simulink model "solenoid_valve_curtain_v1_109"  (R2026a)
settings: Solver=ode15s  StopTime=30  AbsTol=1e-3
values from neighbouring files (symbols this model uses):
  g = 32.174    [RCSMasterCalcs.m]    (also in RCS_180_sweep.m)
  Ixxp = 252099.557 * 0.00029263965    (= 73.7743261256)    [ParabolicNozzle.m]    (also in RCSMasterCalcs.m = 54.4132332957; RCS_180_sweep.m = 12.6144279283)
  mdot_slugs = (Cd * A_actual_m2 * P0_Pa * choke / 0.4536) / g    [RCS_180_sweep.m]
  P0_Pa = P0_abs_psi * 6894.76    (= 1480304.972)    [RCSMasterCalcs.m]    (also in RCS_180_sweep.m = P_psi * 6894.76)
  r_nozzle = 5.0 / 12.0    (= 0.416666666667)    [RCS_180_sweep.m]
libraries: fl_lib x14, nesl_utility x8, ee_lib x2
settings Model: Creator=Lana  LastModifiedBy=Yelkan
settings DebuggingCC: SymbolicDimsDataTypeCodeGenerationDiagnostic=none
settings SimscapeCC: SimscapeNominalValues="[{\"value\":\"1\",\"unit\":\"A\"},{\"value\":\"1\",\"unit\":\"bar\"},{\"value\":\"1\",\"unit\":\"cm^2\"},{\"value\":\"1\",\"unit\":\"cm^3/s\"},{\"value\":\"1\",\"unit\":\"kJ/kg\"},{\"value\":\"1\",\"unit\":\"kW\"},{\"value\":\"1\",\"unit\":\"l\"},{\"value\":\"1\",\"unit\":\"N\"},{\"value\":\"1\",\"unit\":\"N*m\"},{\"value\":\"1\",\"unit\":\"V\"}]"  SimscapeLogSimulationStatistics=on

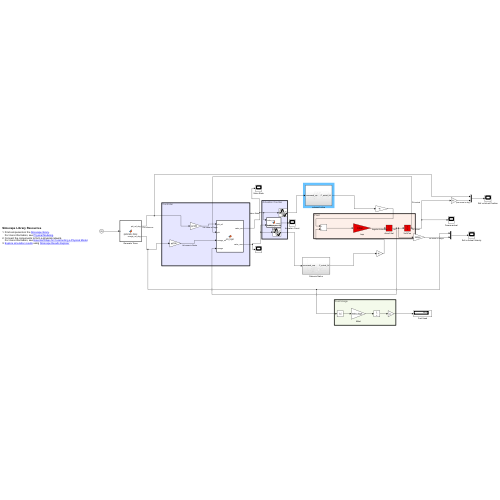
[thumbnail: Simulink's stored preview of the top-level diagram]
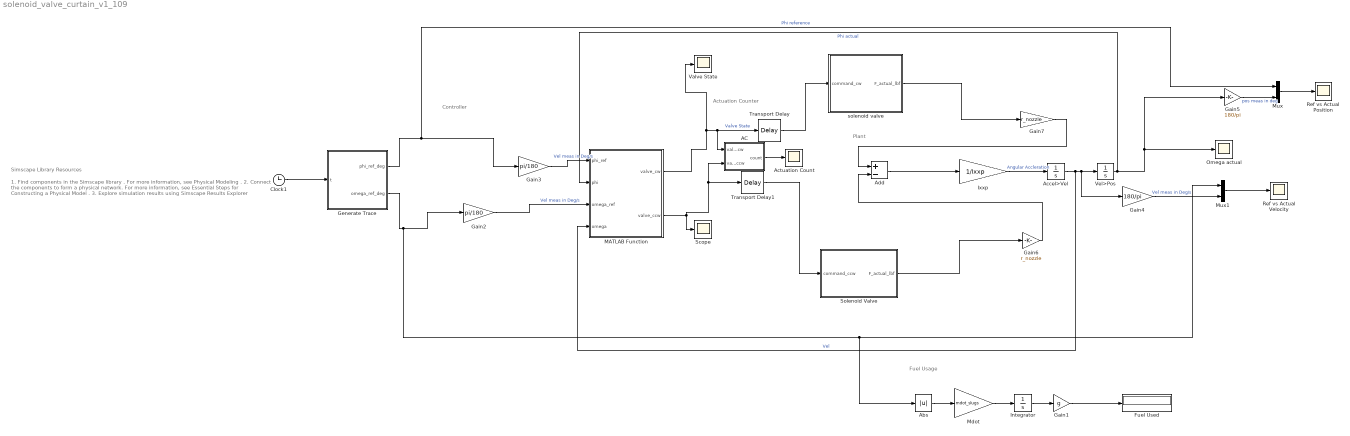
== system solenoid_valve_curtain_v1_109 ==
  note: 1. Find components in the Simscape library .
      | For more information, see Physical Modeling .
      | 2. Connect the components to form a physical network.
      | For more information, see Essential Steps for Constructing a Physical Model .
      | 3. Explore simulation results using Simscape Results Explorer
  note: Simscape Library Resources
  note: Controller
  note: Actuation Counter
  note: Plant
  note: Fuel Usage
  AC : MATLAB Function  TreatAsAtomicUnit=on
  Abs : Abs  SaturateOnIntegerOverflow=off
  Accel>Vel : Integrator
  Actuation Count : Scope
      settings: ActiveDisplayYMinimum=-26.808847302492552  ActiveDisplayYMaximum=50.778884865366138  DataLoggingVariableName=ScopeData3
  Add : Sum  Inputs=+-
  Clock1 : Clock
  Fuel Used : Display
  Gain1 : Gain  Gain=g
  Gain2 : Gain  Gain=pi/180
  Gain3 : Gain  Gain=pi/180
  Gain4 : Gain  Gain=180/pi
  Gain5 : Gain  Gain=180/pi
  Gain6 : Gain  Gain=r_nozzle
  Gain7 : Gain  Gain=r_nozzle
  Generate Trace : MATLAB Function  TreatAsAtomicUnit=on
  Integrator : Integrator
  Ixxp : Gain  Gain=1/Ixxp
  MATLAB Function : MATLAB Function  TreatAsAtomicUnit=on  SystemSampleTime=0.005
  Mdot : Gain  Gain=mdot_slugs
  Mux : Mux  Inputs=2
  Mux1 : Mux  Inputs=2
  Omega actual : Scope
      settings: ActiveDisplayYMinimum=-0.70228346658885066  ActiveDisplayYMaximum=6.3205511992996568  DataLoggingVariableName=ScopeData4
  Ref vs Actual Position : Scope
      settings: ActiveDisplayYMinimum=-60.319230844507317  ActiveDisplayYMaximum=326.94611656087733  DataLoggingVariableName=ScopeData5
  Ref vs Actual Velocity : Scope
      settings: ActiveDisplayYMinimum=-10.640842810110598  ActiveDisplayYMaximum=57.185626811535826
  Scope : Scope
      settings: ActiveDisplayYMinimum=0.21360200383868255  ActiveDisplayYMaximum=1.5917270038386833
  Solenoid Valve : Subsystem
  Transport Delay : TransportDelay  DelayTime=0.005
  Transport Delay1 : TransportDelay  DelayTime=0.005
  Valve State : Scope
      settings: ActiveDisplayYMinimum=-3.9526088666508228  ActiveDisplayYMaximum=5.6960106065109395  DataLoggingVariableName=ScopeData6
  Vel>Pos : Integrator
  solenoid valve : Subsystem
  wires:
  Abs/1 -> Mdot/1
  Mux/1 -> Ref vs Actual Position/1
  Gain4/1 -> Mux1/2  "Vel meas in Deg/s"
  MATLAB Function/1(valve_cw) -> Transport Delay/1, AC/1(valve_cw), Valve State/1  "Valve State"
  Gain5/1 -> Mux/2  "pos meas in deg"
  Integrator/1 -> Gain1/1
  Ixxp/1 -> Accel>Vel/1  "Angular Accleration"
  Mux1/1 -> Ref vs Actual Velocity/1
  Clock1/1 -> Generate Trace/1(t)
  Gain1/1 -> Fuel Used/1
  Vel>Pos/1 -> MATLAB Function/2(phi), Gain5/1, Omega actual/1  "Phi actual"
  Mdot/1 -> Integrator/1
  Accel>Vel/1 -> MATLAB Function/4(omega), Gain4/1, Vel>Pos/1  "Vel"
  MATLAB Function/2(valve_ccw) -> Transport Delay1/1, AC/2(valve_ccw), Scope/1
  Gain7/1 -> Add/1
  Gain6/1 -> Add/2
  Add/1 -> Ixxp/1
  Generate Trace/2(omega_ref_deg) -> Gain2/1, Abs/1, Mux1/1
  Gain3/1 -> MATLAB Function/1(phi_ref)  "Vel meas in Deg/s"
  Gain2/1 -> MATLAB Function/3(omega_ref)  "Vel meas in Deg/s"
  Generate Trace/1(phi_ref_deg) -> Mux/1, Gain3/1  "Phi reference"
  AC/1(count) -> Actuation Count/1
  solenoid valve/1("F_actual_lbf ") -> Gain7/1
  Transport Delay1/1 -> Solenoid Valve/1(command_ccw)
  Solenoid Valve/1(F_actual_lbf) -> Gain6/1
  Transport Delay/1 -> solenoid valve/1("command_cw ")

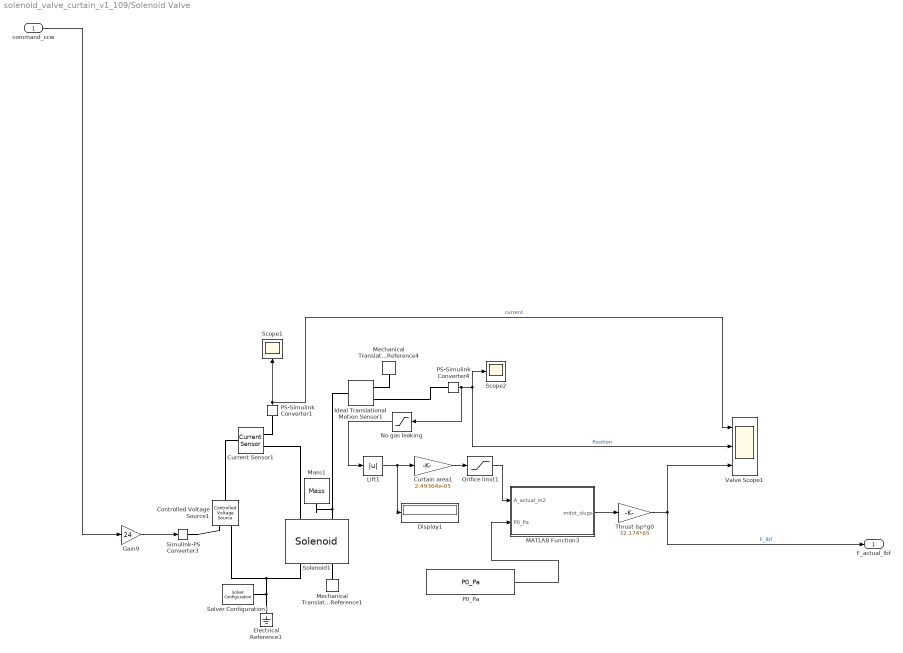
== system solenoid_valve_curtain_v1_109/Solenoid Valve ==
  command_ccw : Inport
  Controlled Voltage Source1 : fl_lib/Electrical/Electrical Sources/Controlled Voltage Source
  Current Sensor1 : fl_lib/Electrical/Electrical Sensors/Current Sensor
  Curtain area1 : Gain  Gain=2.49364e-05
  Display1 : Display
  Electrical Reference1 : fl_lib/Electrical/Electrical Elements/Electrical Reference
  Gain9 : Gain  Gain=24
  Ideal Translational Motion Sensor1 : fl_lib/Mechanical/Mechanical Sensors/Ideal Translational Motion Sensor  reference=foundation.enum.MeasurementReference.difference  acceleration_port=false  velocity_port=false  position_port=true  offset=0 m
  Lift1 : Abs  SaturateOnIntegerOverflow=off
  MATLAB Function3 : MATLAB Function  TreatAsAtomicUnit=on
  Mass1 : fl_lib/Mechanical/Translational Elements/Mass  mass=0.005 kg  num_ports=foundation.enum.numPorts2.one  v_specify=off  v_priority=High  v=0 m/s  v_nominal_specify=off  v_nominal_value=1  v_nominal_unit=m/s  f_specify=off  f_priority=None  f=0 N  f_nominal_specify=off  f_nominal_value=1  f_nominal_unit=N
  Mechanical Translational Reference1 : fl_lib/Mechanical/Translational Elements/Mechanical Translational Reference
  Mechanical Translational Reference4 : fl_lib/Mechanical/Translational Elements/Mechanical Translational Reference
  No gas leaking : Saturate  UpperLimit=0  LowerLimit=-100
  Orifice limit1 : Saturate  UpperLimit=4.94832e-05  LowerLimit=0
  P0_Pa : Constant  Value=P0_Pa
  PS-Simulink Converter1 : nesl_utility/PS-Simulink Converter  PhysicalDomain=network_engine_domain  SubClassName=ps_output  LeftPortType=input  RightPortType=output  PseudoPeriodic=off  Frequencies=[]  VectorFormat=inherit  Unit=A  AffineConversion=off
  PS-Simulink Converter4 : nesl_utility/PS-Simulink Converter  PhysicalDomain=network_engine_domain  SubClassName=ps_output  LeftPortType=input  RightPortType=output  PseudoPeriodic=off  Frequencies=[]  VectorFormat=inherit  Unit=mm  AffineConversion=off
  Scope1 : Scope
      settings: ActiveDisplayYMinimum=-0.033382252757602926  ActiveDisplayYMaximum=0.30044027481842639  DataLoggingVariableName=ScopeData7
  Scope2 : Scope
      settings: ActiveDisplayYMinimum=-7.0487625645709668  ActiveDisplayYMaximum=0.74377868714144668  DataLoggingVariableName=ScopeData10
  Simulink-PS Converter3 : nesl_utility/Simulink-PS Converter  PhysicalDomain=network_engine_domain  SubClassName=ps_input  LeftPortType=input  RightPortType=output  PseudoPeriodic=off  Frequencies=[]  NoiseDistribution=none  NoiseParameters=[]  Unit=V  AffineConversion=off  FilteringAndDerivatives=filter  SimscapeFilterOrder=1  InputFilterTimeConstant=0.001  UdotUserProvided=0
  Solenoid1 : ee_lib/Electromechanical/Mechatronic Actuators/Solenoid  motionDirection=ee.enum.actuators.solenoidDirection.towards  F12=[100, 45] N  X12=[0.1, 1.5] mm  Vdc=24 V  Imax=0.33 A  K=1500 N/m  Xzero=10.3333 mm  lam=5 N*s/m  Mass=0.010 kg  Xmax=7.94 mm  K_endstop=1e6 N/m  D_endstop=500 N*s/m  i_specify=on  i_priority=High  i=0 A  i_nominal_specify=off  i_nominal_value=0.1  i_nominal_unit=A  x_specify=on  x_priority=High  x=7.94 mm  x_nominal_specify=off  x_nominal_value=1  x_nominal_unit=mm  vel_specify=on  vel_priority=Low  vel=0 mm/s  vel_nominal_specify=off  vel_nominal_value=1  vel_nominal_unit=mm/s  F_specify=off  F_priority=High  F=0 N  F_nominal_specify=off  F_nominal_value=100  F_nominal_unit=N  v_L_specify=off  v_L_priority=None  v_L=0 V  v_L_nominal_specify=off  v_L_nominal_value=1  v_L_nominal_unit=V  magnetic_force_specify=off  magnetic_force_priority=None  magnetic_force=0 N  magnetic_force_nominal_specify=off  magnetic_force_nominal_value=1  magnetic_force_nominal_unit=N  alpha=3.93e-3 1/K  Tmeas=25 degC  thermal_mass=100 J/K  temperature_specify=off  temperature_priority=High  temperature=25 degC  temperature_nominal_specify=off  temperature_nominal_value=1  temperature_nominal_unit=degC  Q_specify=off  Q_priority=None  Q=0 W  Q_nominal_specify=off  Q_nominal_value=1  Q_nominal_unit=W
  Solver Configuration1 : nesl_utility/Solver Configuration  PhysicalDomain=network_engine_domain  SubClassName=solver  LeftPortType=input  RightPortType=generic  Tones=[]  Harmonics=[]  SimulateNoise=off  Profile=off  UseLocalSampling=off  EnableSwitchedLinearOptims=on  FrequencyDomain=off  UseCCode=off  RelTol=0.001  AbsTol=0.001  MinStep=1e-09  ToWorkspace=off  RevertToSquareIcSolve=off  NumHomotopyIterations=100  PhasorMode=off  PhasorModeNumHarmonics=1  ConsistencySolver=NEWTON_XTOL_AFTER_FTOL  CanonicalOrdering=UNORDERED  OptimizeIntermediates=UNOPTIMIZED  IndexReductionMethod=DerivativeReplacement  DoDC=off  ResidualTolerance=1e-09  ConsistencyTolSource=GLOBAL  ConsistencyAbsTol=0.001  ConsistencyRelTol=0.001  ConsistencyTolFactor=0.001  UseLocalSolver=off  LocalSolverChoice=NE_BACKWARD_EULER_ADVANCER  ResolveIndetEquations=on  FunctionEvalNumThread=1  LocalSolverSampleTime=0.001  DoFixedCost=off  MaxNonlinIter=3  MaxModeIter=2  ComputeImpulses=off  ImpulseIterations=2  LinearAlgebra=auto  LinearAlgebraNumThread=0  EquationFormulation=NE_TIME_EF  DelaysMemoryBudget=1024  AutomaticFiltering=on  FilteringTimeConstant=0.001  PartitionStorageMethod=AS_NEEDED  PartitionMemoryBudget=1024  PartitionMethod=ROBUST  MultibodyUseLocalSolver=off  MultibodyLocalSolverChoice=ODE1  MultibodyLocalSolverSampleTime=0.001
  Thrust Isp*g0 : Gain  Gain=32.174*65
  Valve Scope1 : Scope  NumInputPorts=3
      settings: ActiveDisplayString=3  ActiveDisplayYMinimum=-1.2268201048220624  ActiveDisplayYMaximum=11.041380943398563  DataLoggingVariableName=ScopeData11
  F_actual_lbf : Outport
  wires:
  PS-Simulink Converter4/1 -> Valve Scope1/2, Scope2/1, No gas leaking/1  "Position"
  Orifice limit1/1 -> MATLAB Function3/1(A_actual_m2)
  Thrust Isp*g0/1 -> F_actual_lbf/1, Valve Scope1/3  "F_lbf"
  command_ccw/1 -> Gain9/1
  MATLAB Function3/1(mdot_slugs) -> Thrust Isp*g0/1
  Gain9/1 -> Simulink-PS Converter3/1
  PS-Simulink Converter1/1 -> Valve Scope1/1, Scope1/1  "current"
  Curtain area1/1 -> Orifice limit1/1
  Lift1/1 -> Display1/1, Curtain area1/1
  No gas leaking/1 -> Lift1/1
  P0_Pa/1 -> MATLAB Function3/2(P0_Pa)
  connections:
  Ideal Translational Motion Sensor1/LConn1 -- Mass1/LConn1 -- Solenoid1/LConn2
  Ideal Translational Motion Sensor1/RConn2 -- PS-Simulink Converter4/LConn1
  Current Sensor1/LConn1 -- Controlled Voltage Source1/LConn1
  Controlled Voltage Source1/RConn2 -- Solenoid1/RConn1 -- Solver Configuration1/RConn1 -- Electrical Reference1/LConn1
  Ideal Translational Motion Sensor1/RConn1 -- Mechanical Translational Reference4/LConn1
  Simulink-PS Converter3/RConn1 -- Controlled Voltage Source1/RConn1
  Current Sensor1/RConn1 -- PS-Simulink Converter1/LConn1
  Solenoid1/LConn1 -- Current Sensor1/RConn2
  Mechanical Translational Reference1/LConn1 -- Solenoid1/RConn2

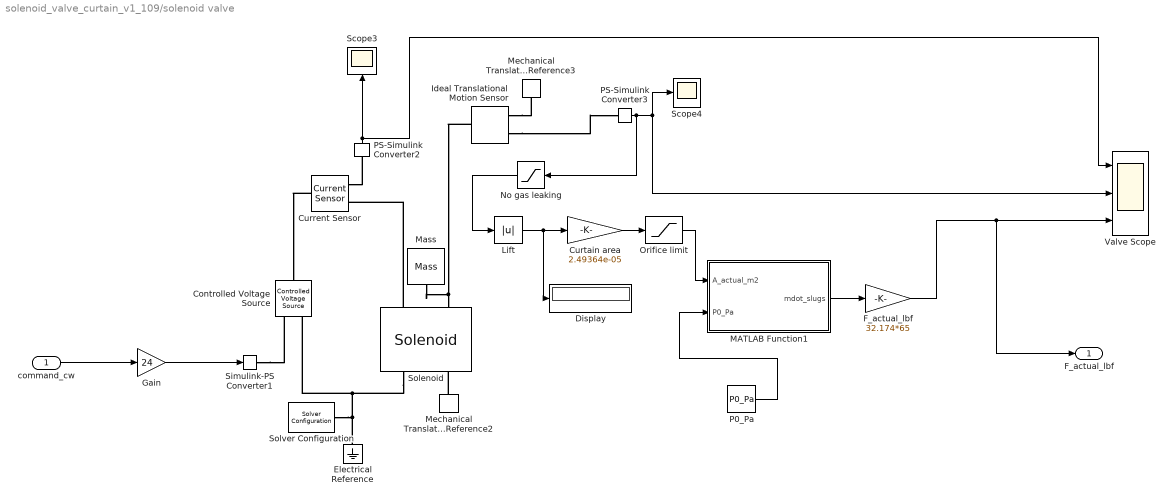
== system solenoid_valve_curtain_v1_109/solenoid valve ==
  "command_cw " : Inport
  Controlled Voltage Source : fl_lib/Electrical/Electrical Sources/Controlled Voltage Source
  Current Sensor : fl_lib/Electrical/Electrical Sensors/Current Sensor
  Curtain area : Gain  Gain=2.49364e-05
  Display : Display
  Electrical Reference : fl_lib/Electrical/Electrical Elements/Electrical Reference
  F_actual_lbf : Gain  Gain=32.174*65
  Gain : Gain  Gain=24
  Ideal Translational Motion Sensor : fl_lib/Mechanical/Mechanical Sensors/Ideal Translational Motion Sensor  reference=foundation.enum.MeasurementReference.difference  acceleration_port=false  velocity_port=false  position_port=true  offset=0 m
  Lift : Abs  SaturateOnIntegerOverflow=off
  MATLAB Function1 : MATLAB Function  TreatAsAtomicUnit=on
  Mass : fl_lib/Mechanical/Translational Elements/Mass  mass=0.005 kg  num_ports=foundation.enum.numPorts2.one  v_specify=off  v_priority=High  v=0 m/s  v_nominal_specify=off  v_nominal_value=1  v_nominal_unit=m/s  f_specify=off  f_priority=None  f=0 N  f_nominal_specify=off  f_nominal_value=1  f_nominal_unit=N
  Mechanical Translational Reference2 : fl_lib/Mechanical/Translational Elements/Mechanical Translational Reference
  Mechanical Translational Reference3 : fl_lib/Mechanical/Translational Elements/Mechanical Translational Reference
  "No gas leaking " : Saturate  UpperLimit=0  LowerLimit=-100
  Orifice limit : Saturate  UpperLimit=4.94832e-05  LowerLimit=0
  P0_Pa : Constant  Value=P0_Pa
  PS-Simulink Converter2 : nesl_utility/PS-Simulink Converter  PhysicalDomain=network_engine_domain  SubClassName=ps_output  LeftPortType=input  RightPortType=output  PseudoPeriodic=off  Frequencies=[]  VectorFormat=inherit  Unit=A  AffineConversion=off
  PS-Simulink Converter3 : nesl_utility/PS-Simulink Converter  PhysicalDomain=network_engine_domain  SubClassName=ps_output  LeftPortType=input  RightPortType=output  PseudoPeriodic=off  Frequencies=[]  VectorFormat=inherit  Unit=mm  AffineConversion=off
  Scope3 : Scope
      settings: ActiveDisplayYMinimum=-0.041230845228280535  ActiveDisplayYMaximum=0.37107760705452486  DataLoggingVariableName=ScopeData8
  Scope4 : Scope
      settings: ActiveDisplayYMinimum=-7.7129135305144487  ActiveDisplayYMaximum=0.25338995146879784  DataLoggingVariableName=ScopeData9
  Simulink-PS Converter1 : nesl_utility/Simulink-PS Converter  PhysicalDomain=network_engine_domain  SubClassName=ps_input  LeftPortType=input  RightPortType=output  PseudoPeriodic=off  Frequencies=[]  NoiseDistribution=none  NoiseParameters=[]  Unit=V  AffineConversion=off  FilteringAndDerivatives=filter  SimscapeFilterOrder=1  InputFilterTimeConstant=0.001  UdotUserProvided=0
  Solenoid : ee_lib/Electromechanical/Mechatronic Actuators/Solenoid  motionDirection=ee.enum.actuators.solenoidDirection.towards  F12=[100, 45] N  X12=[0.1, 1.5] mm  Vdc=24 V  Imax=0.33 A  K=1500 N/m  Xzero=10.3333 mm  lam=5 N*s/m  Mass=0.010 kg  Xmax=7.94 mm  K_endstop=1e6 N/m  D_endstop=500 N*s/m  i_specify=on  i_priority=High  i=0 A  i_nominal_specify=off  i_nominal_value=0.1  i_nominal_unit=A  x_specify=on  x_priority=High  x=7.94 mm  x_nominal_specify=off  x_nominal_value=1  x_nominal_unit=mm  vel_specify=on  vel_priority=Low  vel=0 mm/s  vel_nominal_specify=off  vel_nominal_value=1  vel_nominal_unit=mm/s  F_specify=off  F_priority=High  F=0 N  F_nominal_specify=off  F_nominal_value=100  F_nominal_unit=N  v_L_specify=off  v_L_priority=None  v_L=0 V  v_L_nominal_specify=off  v_L_nominal_value=1  v_L_nominal_unit=V  magnetic_force_specify=off  magnetic_force_priority=None  magnetic_force=0 N  magnetic_force_nominal_specify=off  magnetic_force_nominal_value=1  magnetic_force_nominal_unit=N  alpha=3.93e-3 1/K  Tmeas=25 degC  thermal_mass=100 J/K  temperature_specify=off  temperature_priority=High  temperature=25 degC  temperature_nominal_specify=off  temperature_nominal_value=1  temperature_nominal_unit=degC  Q_specify=off  Q_priority=None  Q=0 W  Q_nominal_specify=off  Q_nominal_value=1  Q_nominal_unit=W
  Solver Configuration : nesl_utility/Solver Configuration  PhysicalDomain=network_engine_domain  SubClassName=solver  LeftPortType=input  RightPortType=generic  Tones=[]  Harmonics=[]  SimulateNoise=off  Profile=off  UseLocalSampling=off  EnableSwitchedLinearOptims=on  FrequencyDomain=off  UseCCode=off  RelTol=0.001  AbsTol=0.001  MinStep=1e-09  ToWorkspace=off  RevertToSquareIcSolve=off  NumHomotopyIterations=100  PhasorMode=off  PhasorModeNumHarmonics=1  ConsistencySolver=NEWTON_XTOL_AFTER_FTOL  CanonicalOrdering=UNORDERED  OptimizeIntermediates=UNOPTIMIZED  IndexReductionMethod=DerivativeReplacement  DoDC=off  ResidualTolerance=1e-09  ConsistencyTolSource=GLOBAL  ConsistencyAbsTol=0.001  ConsistencyRelTol=0.001  ConsistencyTolFactor=0.001  UseLocalSolver=off  LocalSolverChoice=NE_BACKWARD_EULER_ADVANCER  ResolveIndetEquations=on  FunctionEvalNumThread=1  LocalSolverSampleTime=0.001  DoFixedCost=off  MaxNonlinIter=3  MaxModeIter=2  ComputeImpulses=off  ImpulseIterations=2  LinearAlgebra=auto  LinearAlgebraNumThread=0  EquationFormulation=NE_TIME_EF  DelaysMemoryBudget=1024  AutomaticFiltering=on  FilteringTimeConstant=0.001  PartitionStorageMethod=AS_NEEDED  PartitionMemoryBudget=1024  PartitionMethod=ROBUST  MultibodyUseLocalSolver=off  MultibodyLocalSolverChoice=ODE1  MultibodyLocalSolverSampleTime=0.001
  Valve Scope : Scope  NumInputPorts=3
      settings: ActiveDisplayYMinimum=-0.052528651859260825  ActiveDisplayYMaximum=0.40204141678253213  DataLoggingVariableName=ScopeData2
  "F_actual_lbf " : Outport
  wires:
  PS-Simulink Converter2/1 -> Valve Scope/1, Scope3/1
  F_actual_lbf/1 -> "F_actual_lbf "/1, Valve Scope/3
  "command_cw "/1 -> Gain/1
  PS-Simulink Converter3/1 -> Valve Scope/2, Scope4/1, "No gas leaking "/1
  Lift/1 -> Display/1, Curtain area/1
  Curtain area/1 -> Orifice limit/1
  Orifice limit/1 -> MATLAB Function1/1(A_actual_m2)
  Gain/1 -> Simulink-PS Converter1/1
  MATLAB Function1/1(mdot_slugs) -> F_actual_lbf/1
  "No gas leaking "/1 -> Lift/1
  P0_Pa/1 -> MATLAB Function1/2(P0_Pa)
  connections:
  Ideal Translational Motion Sensor/RConn1 -- Mechanical Translational Reference3/LConn1
  Controlled Voltage Source/RConn2 -- Solenoid/RConn1 -- Solver Configuration/RConn1 -- Electrical Reference/LConn1
  Ideal Translational Motion Sensor/RConn2 -- PS-Simulink Converter3/LConn1
  Ideal Translational Motion Sensor/LConn1 -- Mass/LConn1 -- Solenoid/LConn2
  Simulink-PS Converter1/RConn1 -- Controlled Voltage Source/RConn1
  Current Sensor/RConn1 -- PS-Simulink Converter2/LConn1
  Mechanical Translational Reference2/LConn1 -- Solenoid/RConn2
  Current Sensor/LConn1 -- Controlled Voltage Source/LConn1
  Solenoid/LConn1 -- Current Sensor/RConn2

== matlab function solenoid_valve_curtain_v1_109/Generate Trace ==
  data: t input; phi_ref_deg output; omega_ref_deg output
function [phi_ref_deg, omega_ref_deg] = generate_trace(t)
    start_time = 1.0;
    duration = 10.0;
    target_angle = 180.0;
    
    if t < start_time
        phi_ref_deg = 0;
        omega_ref_deg = 0;
elseif t <= (start_time + duration)
    phi_ref_deg   = (target_angle/duration) * (t - start_time);
    omega_ref_deg = target_angle/duration;
    else
        phi_ref_deg = target_angle;
        omega_ref_deg = 0;
    end
end

== matlab function solenoid_valve_curtain_v1_109/MATLAB Function ==
  settings: updateMethod=DISCRETE
  data: phi_ref input; valve_cw output; valve_ccw output; phi input; omega_ref input; omega input
function [valve_cw, valve_ccw] = rcs_logic(phi_ref, phi, omega_ref, omega)
% Schmitt-trigger valve logic with minimum pulse time.
% Matches RCS_180_sweep.m exactly.
%
% Inputs:
%   phi_ref   - target angle (rad)
%   phi       - actual angle (rad)
%   omega_ref - target angular rate (rad/s)
%   omega     - actual angular rate (rad/s)
% Outputs:
%   valve_cw  - 1 when the clockwise thruster should fire, else 0
%   valve_ccw - 1 when the counter-clockwise thruster should fire, else 0

    % persistent variables keep their value between time steps
    persistent valve_state pulse_timer

    % first time this runs, initialize everything to zero
    if isempty(valve_state)
        valve_state  = 0;
        pulse_timer  = 0;
    end

    % --- Controller gains (match the script) ---
    Kp = 1;
    Kd = 0.5;

    % --- Schmitt trigger parameters (match the script) ---
    deadzone       = 0.02;
    hysteresis     = 0.01;
    min_pulse_time = 0.10;
    dt             = 0.005;   % must match this block's fixed sample time

    % --- PD control effort ---
    error_phi     = phi_ref - phi;
    error_omega   = omega_ref - omega;
    control_effort = (Kp * error_phi) + (Kd * error_omega);

    % --- Minimum pulse timer countdown ---
    if pulse_timer > 0
        pulse_timer = pulse_timer - dt;

    else
        % --- Schmitt trigger state machine ---
        if valve_state == 0
            if control_effort > deadzone
                valve_state = 1;
                pulse_timer = min_pulse_time;
            elseif control_effort < -deadzone
                valve_state = -1;
                pulse_timer = min_pulse_time;
            end

        elseif valve_state == 1
            if control_effort < (deadzone - hysteresis)
                valve_state = 0;
            end

        elseif valve_state == -1
            if control_effort > -(deadzone - hysteresis)
                valve_state = 0;
            end
        end
    end

    % --- Convert signed valve_state into two separate 0/1 outputs ---
    valve_cw  = double(valve_state == 1);
    valve_ccw = double(valve_state == -1);

end

== matlab function solenoid_valve_curtain_v1_109/AC ==
  data: valve_cw input; count output; valve_ccw input
function count = actuation_counter(valve_cw, valve_ccw)
% Counts a "firing" each time a thruster turns ON from OFF.
% Inputs:
%   valve_cw  - 1 when the clockwise thruster is firing, else 0
%   valve_ccw - 1 when the counter-clockwise thruster is firing, else 0
% Output:
%   count - running total of firings so far

    % persistent variables keep their value between time steps
    persistent total prev_cw prev_ccw

    % first time this runs, initialize everything to zero
    if isempty(total)
        total   = 0;
        prev_cw  = 0;
        prev_ccw = 0;
    end

    % a "firing" is a transition from 0 -> 1 on either valve
    cw_just_turned_on  = (valve_cw  == 1) && (prev_cw  == 0);
    ccw_just_turned_on = (valve_ccw == 1) && (prev_ccw == 0);

    if cw_just_turned_on || ccw_just_turned_on
        total = total + 1;
    end

    % remember this step's values for next time
    prev_cw  = valve_cw;
    prev_ccw = valve_ccw;

    count = total;
end

== matlab function solenoid_valve_curtain_v1_109/solenoid valve/MATLAB Function1 ==
  data: A_actual_m2 input; mdot_slugs output; P0_Pa input
function mdot_slugs = fcn(A_actual_m2,P0_Pa)

gamma = 1.4; R = 296.8; T0 = 300; g = 32.174; Cd = 0.9;
choke = sqrt(gamma/(R*T0)) * (2/(gamma+1))^((gamma+1)/(2*(gamma-1)));
mdot_slugs = (Cd * A_actual_m2 * P0_Pa * choke / 0.4536) / g;

== matlab function solenoid_valve_curtain_v1_109/Solenoid Valve/MATLAB Function3 ==
  data: A_actual_m2 input; mdot_slugs output; P0_Pa input
function mdot_slugs = fcn(A_actual_m2,P0_Pa)

gamma = 1.4; R = 296.8; T0 = 300; g = 32.174; Cd = 0.9;
choke = sqrt(gamma/(R*T0)) * (2/(gamma+1))^((gamma+1)/(2*(gamma-1)));
mdot_slugs = (Cd * A_actual_m2 * P0_Pa * choke / 0.4536) / g;
